simulink model "State_Space_Eigenvalue"  (R2026b)
settings: Solver=VariableStepAuto
undefined symbols (not defined in the file): A, B, C, D, F, x0
settings Model: Creator=Arjun  LastModifiedBy=Arjun

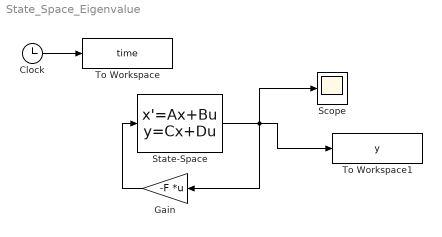
== system State_Space_Eigenvalue ==
  Clock : Clock
  Gain : Gain  Gain=-F  Multiplication=Matrix(K*u)
  Scope : Scope
      settings: ActiveDisplayYMinimum=-1  ActiveDisplayYMaximum=1
  State-Space : StateSpace  A=A  B=B  C=C  D=D  InitialCondition=x0
  To Workspace : ToWorkspace  VariableName=time  SampleTime=-1
  To Workspace1 : ToWorkspace  VariableName=y  SampleTime=-1
  wires:
  Clock/1 -> To Workspace/1
  State-Space/1 -> Scope/1, Gain/1, To Workspace1/1
  Gain/1 -> State-Space/1
